simulink model "fulladder"  (R2022b)
settings: Solver=VariableStepAuto  StartTime=0.0  StopTime=10.0  RelTol=1e-3
undefined symbols (not defined in the file): s0, s1, s2, s3
settings Model: Creator=shaibalsaha  LastModifiedBy=shaibalsaha

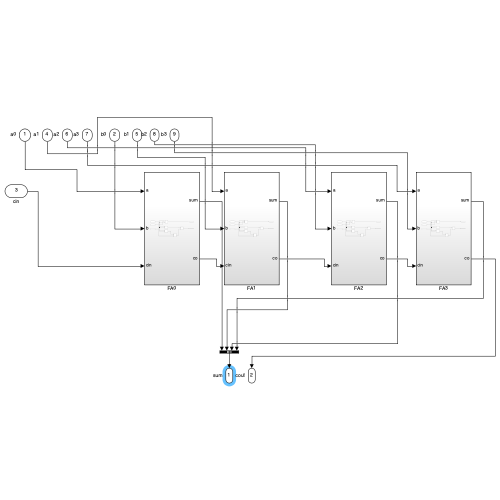
[thumbnail: Simulink's stored preview of the top-level diagram]
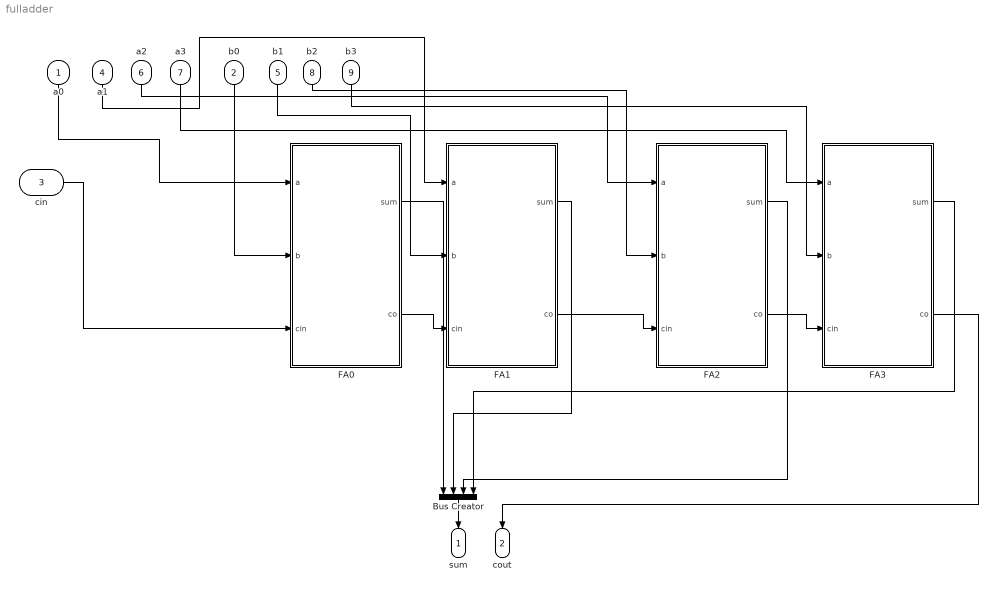
== system fulladder ==
  a0 : Inport
  b0 : Inport  Port=2
  cin : Inport  Port=3
  a1 : Inport  Port=4
  b1 : Inport  Port=5
  a2 : Inport  Port=6
  a3 : Inport  Port=7
  b2 : Inport  Port=8
  b3 : Inport  Port=9
  Bus Creator : BusCreator  Inputs=s0,s1,s2,s3
  FA0 : Subsystem
  FA1 : Subsystem
  FA2 : Subsystem
  FA3 : Subsystem
  sum : Outport  VectorParamsAs1DForOutWhenUnconnected=off
  cout : Outport  Port=2  VectorParamsAs1DForOutWhenUnconnected=off
  wires:
  a0/1 -> FA0/1(a)
  b0/1 -> FA0/2(b)
  cin/1 -> FA0/3(cin)
  b1/1 -> FA1/2(b)
  FA1/1(sum) -> Bus Creator/2
  a1/1 -> FA1/1(a)
  FA0/2(co) -> FA1/3(cin)
  FA1/2(co) -> FA2/3(cin)
  a2/1 -> FA2/1(a)
  b2/1 -> FA2/2(b)
  FA2/1(sum) -> Bus Creator/3
  FA2/2(co) -> FA3/3(cin)
  b3/1 -> FA3/2(b)
  a3/1 -> FA3/1(a)
  FA3/1(sum) -> Bus Creator/4
  FA3/2(co) -> cout/1
  FA0/1(sum) -> Bus Creator/1
  Bus Creator/1 -> sum/1

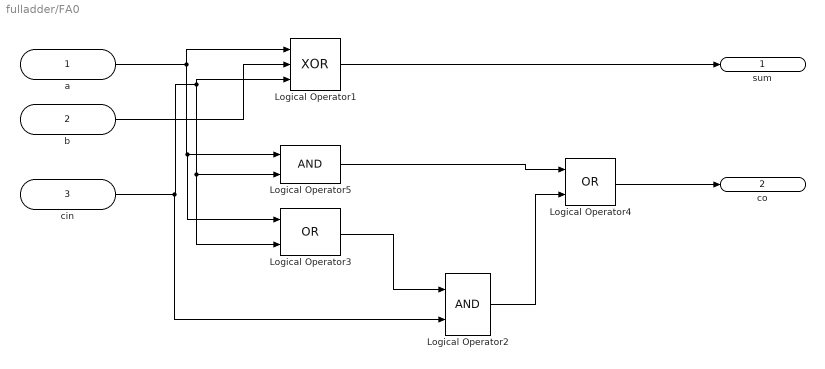
== system fulladder/FA0 ==
  a : Inport
  b : Inport  Port=2
  cin : Inport  Port=3
  Logical Operator1 : Logic  Operator=XOR  Inputs=3  AllPortsSameDT=off  OutDataTypeStr=boolean
  Logical Operator2 : Logic  AllPortsSameDT=off  OutDataTypeStr=boolean
  Logical Operator3 : Logic  Operator=OR  AllPortsSameDT=off  OutDataTypeStr=boolean
  Logical Operator4 : Logic  Operator=OR  AllPortsSameDT=off  OutDataTypeStr=boolean
  Logical Operator5 : Logic  AllPortsSameDT=off  OutDataTypeStr=boolean
  sum : Outport  VectorParamsAs1DForOutWhenUnconnected=off
  co : Outport  Port=2  VectorParamsAs1DForOutWhenUnconnected=off
  wires:
  Logical Operator4/1 -> co/1
  b/1 -> Logical Operator1/2
  cin/1 -> Logical Operator2/2, Logical Operator1/3, Logical Operator5/2, Logical Operator3/2
  Logical Operator3/1 -> Logical Operator2/1
  Logical Operator5/1 -> Logical Operator4/1
  a/1 -> Logical Operator1/1, Logical Operator5/1, Logical Operator3/1
  Logical Operator2/1 -> Logical Operator4/2
  Logical Operator1/1 -> sum/1

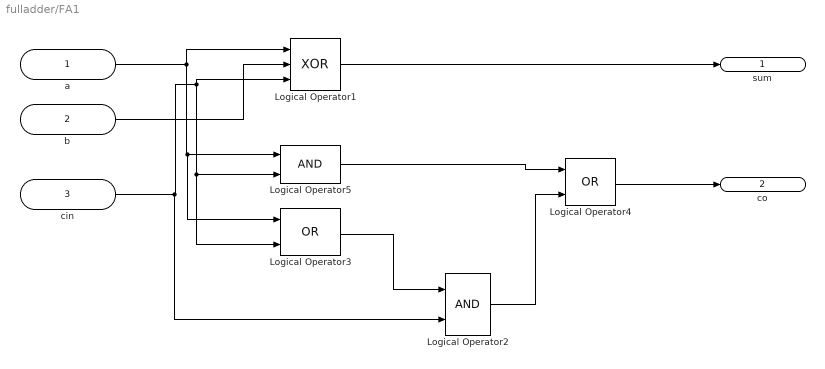
== system fulladder/FA1 ==
  a : Inport
  b : Inport  Port=2
  cin : Inport  Port=3
  Logical Operator1 : Logic  Operator=XOR  Inputs=3  AllPortsSameDT=off  OutDataTypeStr=boolean
  Logical Operator2 : Logic  AllPortsSameDT=off  OutDataTypeStr=boolean
  Logical Operator3 : Logic  Operator=OR  AllPortsSameDT=off  OutDataTypeStr=boolean
  Logical Operator4 : Logic  Operator=OR  AllPortsSameDT=off  OutDataTypeStr=boolean
  Logical Operator5 : Logic  AllPortsSameDT=off  OutDataTypeStr=boolean
  sum : Outport  VectorParamsAs1DForOutWhenUnconnected=off
  co : Outport  Port=2  VectorParamsAs1DForOutWhenUnconnected=off
  wires:
  Logical Operator4/1 -> co/1
  b/1 -> Logical Operator1/2
  cin/1 -> Logical Operator2/2, Logical Operator1/3, Logical Operator5/2, Logical Operator3/2
  Logical Operator3/1 -> Logical Operator2/1
  Logical Operator5/1 -> Logical Operator4/1
  a/1 -> Logical Operator1/1, Logical Operator5/1, Logical Operator3/1
  Logical Operator2/1 -> Logical Operator4/2
  Logical Operator1/1 -> sum/1

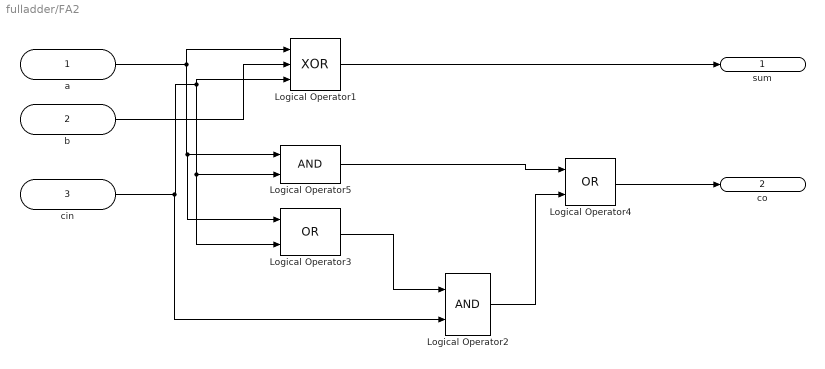
== system fulladder/FA2 ==
  a : Inport
  b : Inport  Port=2
  cin : Inport  Port=3
  Logical Operator1 : Logic  Operator=XOR  Inputs=3  AllPortsSameDT=off  OutDataTypeStr=boolean
  Logical Operator2 : Logic  AllPortsSameDT=off  OutDataTypeStr=boolean
  Logical Operator3 : Logic  Operator=OR  AllPortsSameDT=off  OutDataTypeStr=boolean
  Logical Operator4 : Logic  Operator=OR  AllPortsSameDT=off  OutDataTypeStr=boolean
  Logical Operator5 : Logic  AllPortsSameDT=off  OutDataTypeStr=boolean
  sum : Outport  VectorParamsAs1DForOutWhenUnconnected=off
  co : Outport  Port=2  VectorParamsAs1DForOutWhenUnconnected=off
  wires:
  Logical Operator4/1 -> co/1
  b/1 -> Logical Operator1/2
  cin/1 -> Logical Operator2/2, Logical Operator1/3, Logical Operator5/2, Logical Operator3/2
  Logical Operator3/1 -> Logical Operator2/1
  Logical Operator5/1 -> Logical Operator4/1
  a/1 -> Logical Operator1/1, Logical Operator5/1, Logical Operator3/1
  Logical Operator2/1 -> Logical Operator4/2
  Logical Operator1/1 -> sum/1

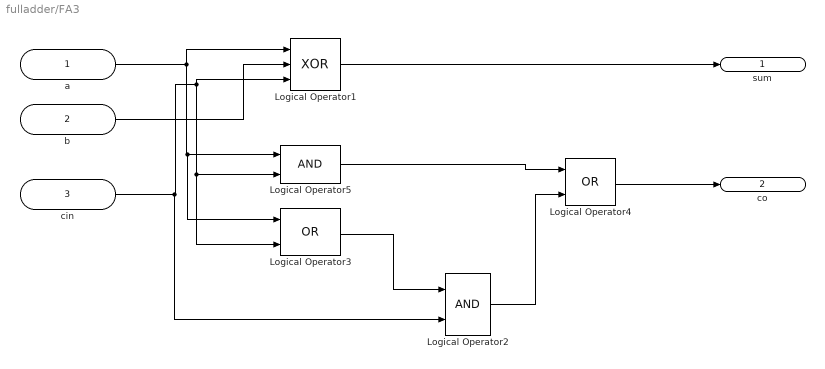
== system fulladder/FA3 ==
  a : Inport
  b : Inport  Port=2
  cin : Inport  Port=3
  Logical Operator1 : Logic  Operator=XOR  Inputs=3  AllPortsSameDT=off  OutDataTypeStr=boolean
  Logical Operator2 : Logic  AllPortsSameDT=off  OutDataTypeStr=boolean
  Logical Operator3 : Logic  Operator=OR  AllPortsSameDT=off  OutDataTypeStr=boolean
  Logical Operator4 : Logic  Operator=OR  AllPortsSameDT=off  OutDataTypeStr=boolean
  Logical Operator5 : Logic  AllPortsSameDT=off  OutDataTypeStr=boolean
  sum : Outport  VectorParamsAs1DForOutWhenUnconnected=off
  co : Outport  Port=2  VectorParamsAs1DForOutWhenUnconnected=off
  wires:
  Logical Operator4/1 -> co/1
  b/1 -> Logical Operator1/2
  cin/1 -> Logical Operator2/2, Logical Operator1/3, Logical Operator5/2, Logical Operator3/2
  Logical Operator3/1 -> Logical Operator2/1
  Logical Operator5/1 -> Logical Operator4/1
  a/1 -> Logical Operator1/1, Logical Operator5/1, Logical Operator3/1
  Logical Operator2/1 -> Logical Operator4/2
  Logical Operator1/1 -> sum/1
